simulink model "a"  (R2025b)
settings: Solver=VariableStepAuto  StartTime=0.0  StopTime=50  RelTol=1e-3
values from neighbouring files (symbols this model uses):
  Cd_mach = data_flight.CD    [load_aero.m]
  CnA_mach = data_flight.("CNalpha (0 to 4 deg) (per rad)")    [load_aero.m]
  Cp_inches_mach = data_flight.CP    [load_aero.m]
  Mach_vec = data_flight.Mach    [load_aero.m]
  thrust_force_vec = eng_data(:, 2)    [load_aero.m]
  thrust_time_vec = eng_data(:, 1)    [load_aero.m]
libraries: simulink_extras x6, aerolibasang x3, slpidlib x3, aerolibwind2 x2, aerolibanim x1, aerolibatmos2 x1, simulink x1
settings Model: Creator=anth  LastModifiedBy=anth

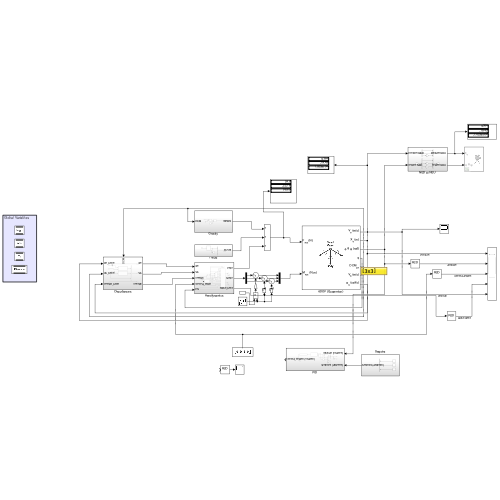
[thumbnail: Simulink's stored preview of the top-level diagram]
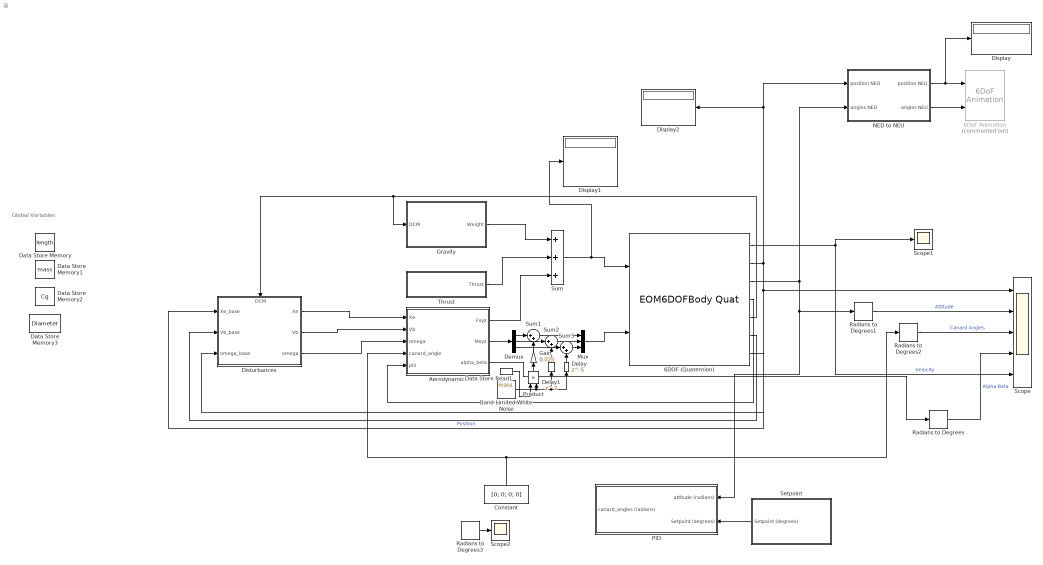
== system a ==
  note: Global Variables
  6DOF (Quaternion) : EOM6DOFBodyQuat  pm_0=[0.5 0.5 -0.5]  mass_0=5  inertia=[0.06 0 0; 0 0.06 0; 0 0 0.00056]
  6DoF Animation : aerolibanim/6DoF Animation  Commented=on  u1=[-4000 4000 -2000 2000 -5000000 4000000]  u2=0.1  u3=2  u4=[-1000 0 -1000]  u5=Fly alongside  u6=[40 5 -40]  u7=10  u8=on
  Aerodynamics : Subsystem
  Band-Limited White Noise : simulink/Sources/Band-Limited White Noise  Cov=[0.1]  Ts=0.1  seed=[23341]
  Constant : Constant  Value=[0; 0; 0; 0]
  Data Store Memory : DataStoreMemory  DataStoreName=length  WriteAfterWriteMsg=warning  InitialValue=1.524  ShowAdditionalParam=off
  Data Store Memory1 : DataStoreMemory  DataStoreName=mass  WriteAfterWriteMsg=warning  InitialValue=5  ShowAdditionalParam=off
  Data Store Memory2 : DataStoreMemory  DataStoreName=Cg  WriteAfterWriteMsg=warning  InitialValue=0.911682  ShowAdditionalParam=off
  Data Store Memory3 : DataStoreMemory  DataStoreName=Diameter  WriteAfterWriteMsg=warning  InitialValue=0.1016  ShowAdditionalParam=off
  Data Store Read1 : DataStoreRead  DataStoreName=mass  IndexOptions=Index vector (dialog)  Indices=1  OutputSizes=1
  Delay : Delay  DelayLength=5
  Delay1 : Delay
  Demux : Demux  Outputs=3
  Display : Display
  Display1 : Display
  Display2 : Display
  Disturbances : Subsystem
      settings: PortSchema="{\"entries\":[{\"content\":{\"sides\":[{\"content\":{\"connectorIds\":[\"In1\",\"In2\",\"In3\"]},\"type\":\"ConnectorPlacement.EquallySpacedRectSide\",\"uuid\":\"32f54cef-b4cb-4256-8316-c563039928ca\"},{\"content\":{\"connectorIds\":[\"Out1\",\"Out2\",\"Out3\"],\"side\":\"RIGHT\"},\"type\":\"ConnectorPlacement.EquallySpacedRectSide\",\"uuid\":\"bb564e65-4080-434d-8692-2d229c22ab5f\"},{\"content\":{\"connectorIds\":[\"In4\"],\"side\":\"TOP\"},\"type\":\"ConnectorPlacement.EquallySpacedRectSide\",\"uuid\":\"6318908c-0300-48fa-8f39-f8088bf31443\"}]},\"type\":\"ConnectorPlacement.EquallySpacedConnector\",\"uuid\":\"3467b8b9-b405-4e5c-95ab-dad331d67992\"}],\"packageUris\":[\"http://schema.mathworks.com/mf0/Connector/R2020b\"],\"version\":\"1.0\"}"
  Gain : Gain  Gain=0.025
  Gravity : Subsystem
  Mux : Mux  Inputs=3
  NED to NEU : Subsystem
  PID : Subsystem
  Product : Product
  Radians to Degrees{,1..3} (4 alike) : simulink_extras/Transformations/Radians to Degrees
  Scope : Scope  NumInputPorts=5
      settings: ActiveDisplayYMinimum=-186.34807824721173  ActiveDisplayYMaximum=22699.188645995033  DataLoggingVariableName=ScopeData7
  Scope1 : Scope
      settings: DataLoggingVariableName=ScopeData8
  Scope2 : Scope
      settings: ActiveDisplayYMinimum=-0.21482274425849368  ActiveDisplayYMaximum=0.19778218203879105  DataLoggingVariableName=ScopeData10
  Setpoint : Subsystem
  Sum : Sum  Inputs=+++
  Sum1 : Sum  Inputs=|++
  Sum2 : Sum  Inputs=|++
  Sum3 : Sum  Inputs=|++
  Thrust : Subsystem
  wires:
  Sum/1 -> Display1/1, 6DOF (Quaternion)/1
  Aerodynamics/1(Fxyz) -> Sum/3
  Aerodynamics/2(Mxyz) -> Demux/1
  Mux/1 -> 6DOF (Quaternion)/2
  Sum3/1 -> Mux/3
  Sum2/1 -> Mux/2
  Sum1/1 -> Mux/1
  Demux/1 -> Sum1/1
  Demux/2 -> Sum2/1
  Demux/3 -> Sum3/1
  Band-Limited White Noise/1 -> Product/2, Delay1/1, Delay/1
  Gain/1 -> Sum1/2
  Thrust/1(Thrust) -> Sum/2
  Gravity/1(Weight) -> Sum/1
  NED to NEU/1(position NEU) -> Display/1, 6DoF Animation/1
  NED to NEU/2(angles NEU) -> 6DoF Animation/2
  Setpoint/1(Setpoint (degrees)) -> PID/2(Setpoint (degrees))
  Disturbances/2(Vb) -> Aerodynamics/2(Vb)
  Disturbances/1(Xe) -> Aerodynamics/1(Xe)
  Disturbances/3(omega) -> Aerodynamics/3(omega)
  6DOF (Quaternion)/7 -> Disturbances/3(omega_base)
  6DOF (Quaternion)/6 -> Disturbances/2(Vb_base)
  6DOF (Quaternion)/2 -> NED to NEU/1(position NED), Display2/1, Scope/1, Disturbances/1(Xe_base)  "Position"
  6DOF (Quaternion)/5 -> Disturbances/4(DCM), Gravity/1(DCM)
  6DOF (Quaternion)/4 -> Aerodynamics/5(phi)
  Aerodynamics/3(alpha_beta) -> Radians to Degrees/1
  Radians to Degrees/1 -> Scope/4  "Alpha Beta"
  6DOF (Quaternion)/1 -> Scope/5, Scope1/1  "Velocity"
  Radians to Degrees1/1 -> Scope/2  "Attitude"
  6DOF (Quaternion)/3 -> NED to NEU/2(angles NED), PID/1(attitude (radians)), Radians to Degrees1/1
  Radians to Degrees2/1 -> Scope/3  "Canard Angles"
  Delay1/1 -> Sum2/2
  Delay/1 -> Sum3/2
  Radians to Degrees3/1 -> Scope2/1
  Constant/1 -> Radians to Degrees2/1, Aerodynamics/4(canard_angle)
  Product/1 -> Gain/1
  Data Store Read1/1 -> Product/1

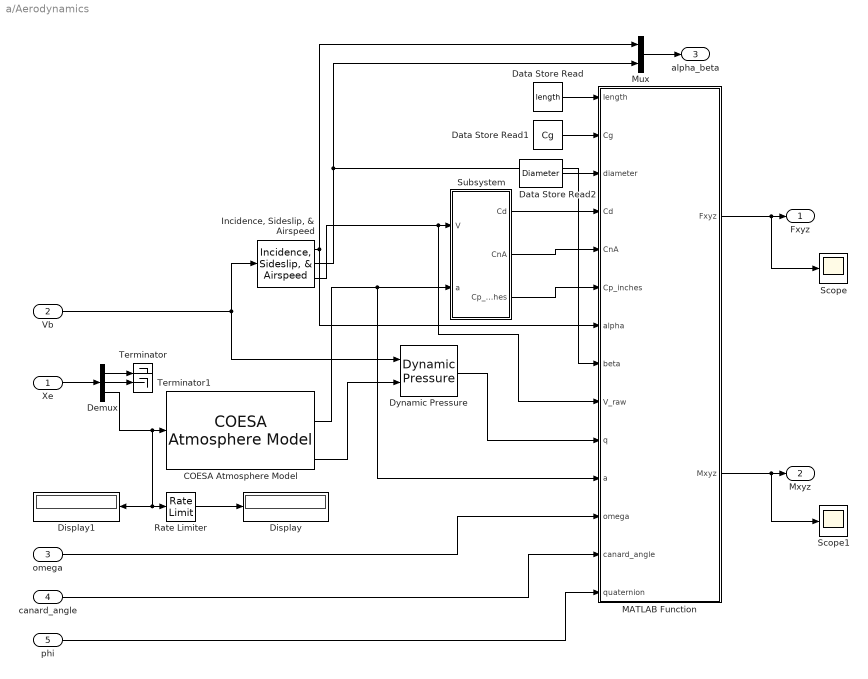
== system a/Aerodynamics ==
  Xe : Inport
  Vb : Inport  Port=2
  omega : Inport  Port=3
  canard_angle : Inport  Port=4
  phi : Inport  Port=5
  COESA Atmosphere Model : aerolibatmos2/COESA Atmosphere Model  units=Metric (MKS)  spec=1976 COESA-extended U.S. Standard Atmosphere  model=Profile  profile_var=High temperature  profile_percent=1%  profile_alt=5 km (16404 ft)  envelope_var=High temperature  envelope_percent=1%  action=Warning
  Data Store Read : DataStoreRead  DataStoreName=length  IndexOptions=Index vector (dialog)  Indices=1  OutputSizes=1
  Data Store Read1 : DataStoreRead  DataStoreName=Cg  IndexOptions=Index vector (dialog)  Indices=1  OutputSizes=1
  Data Store Read2 : DataStoreRead  DataStoreName=Diameter  IndexOptions=Index vector (dialog)  Indices=1  OutputSizes=1
  Demux : Demux  Outputs=3
  Display : Display
  Display1 : Display
  Dynamic Pressure : aerolibasang/Dynamic Pressure
  "Incidence, Sideslip, & Airspeed" : aerolibasang/Incidence, Sideslip, & Airspeed
  MATLAB Function : MATLAB Function  TreatAsAtomicUnit=on
  Mux : Mux  Inputs=2
  Rate Limiter : RateLimiter  RisingSlewLimit=inf  FallingSlewLimit=0  SampleTimeMode=inherited
  Scope : Scope
      settings: ActiveDisplayYMinimum=-4834.811497564544  ActiveDisplayYMaximum=1699.3324805277052
  Scope1 : Scope
      settings: DataLoggingVariableName=ScopeData2
  Subsystem : Subsystem
  Terminator : Terminator
  Terminator1 : Terminator
  Fxyz : Outport
  Mxyz : Outport  Port=2
  alpha_beta : Outport  Port=3
  wires:
  Xe/1 -> Demux/1
  Demux/1 -> Terminator/1
  Demux/2 -> Terminator1/1
  Demux/3 -> Display1/1, Rate Limiter/1, COESA Atmosphere Model/1
  Rate Limiter/1 -> Display/1
  COESA Atmosphere Model/4 -> Dynamic Pressure/2
  Vb/1 -> "Incidence, Sideslip, & Airspeed"/1, Dynamic Pressure/1
  "Incidence, Sideslip, & Airspeed"/3 -> MATLAB Function/9(V_raw), Subsystem/1(V)
  COESA Atmosphere Model/2 -> Subsystem/2(a), MATLAB Function/11(a)
  Mux/1 -> alpha_beta/1
  "Incidence, Sideslip, & Airspeed"/1 -> MATLAB Function/7(alpha), Mux/1
  "Incidence, Sideslip, & Airspeed"/2 -> MATLAB Function/8(beta), Mux/2
  MATLAB Function/1(Fxyz) -> Scope/1, Fxyz/1
  MATLAB Function/2(Mxyz) -> Scope1/1, Mxyz/1
  Subsystem/1(Cd) -> MATLAB Function/4(Cd)
  Subsystem/2(CnA) -> MATLAB Function/5(CnA)
  Subsystem/3(Cp_inches) -> MATLAB Function/6(Cp_inches)
  Dynamic Pressure/1 -> MATLAB Function/10(q)
  omega/1 -> MATLAB Function/12(omega)
  canard_angle/1 -> MATLAB Function/13(canard_angle)
  phi/1 -> MATLAB Function/14(quaternion)
  Data Store Read1/1 -> MATLAB Function/2(Cg)
  Data Store Read2/1 -> MATLAB Function/3(diameter)
  Data Store Read/1 -> MATLAB Function/1(length)

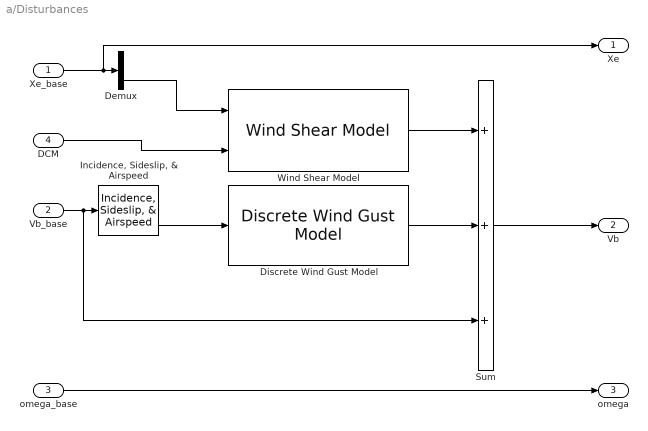
== system a/Disturbances ==
  Xe_base : Inport
  Vb_base : Inport  Port=2
  omega_base : Inport  Port=3
  DCM : Inport  Port=4
  Demux : Demux  Outputs=3
  Discrete Wind Gust Model : aerolibwind2/Discrete Wind Gust Model  units=Metric (MKS)  Gx=on  Gy=on  Gz=on  t_0=5  d_m=[120 120 80]  v_m=[3.5 3.5 3.0]
  "Incidence, Sideslip, & Airspeed" : aerolibasang/Incidence, Sideslip, & Airspeed
  Sum : Sum  Inputs=+++
  Wind Shear Model : aerolibwind2/Wind Shear Model  units=Metric (MKS)  phase=Category C - Terminal Flight Phase  W_20=15  Wdeg=0
  Xe : Outport
  Vb : Outport  Port=2
  omega : Outport  Port=3
  wires:
  omega_base/1 -> omega/1
  Vb_base/1 -> Sum/3, "Incidence, Sideslip, & Airspeed"/1
  "Incidence, Sideslip, & Airspeed"/3 -> Discrete Wind Gust Model/1
  Discrete Wind Gust Model/1 -> Sum/2
  Wind Shear Model/1 -> Sum/1
  Sum/1 -> Vb/1
  DCM/1 -> Wind Shear Model/2
  Demux/3 -> Wind Shear Model/1
  Xe_base/1 -> Xe/1, Demux/1

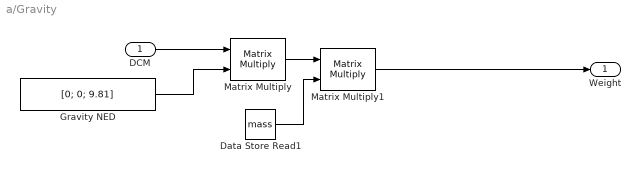
== system a/Gravity ==
  DCM : Inport
  Data Store Read1 : DataStoreRead  DataStoreName=mass  IndexOptions=Index vector (dialog)  Indices=1  OutputSizes=1
  Gravity NED : Constant  Value=[0; 0; 9.81]
  Matrix Multiply : Product  Multiplication=Matrix(*)
  Matrix Multiply1 : Product  Multiplication=Matrix(*)
  Weight : Outport
  wires:
  DCM/1 -> Matrix Multiply/1
  Gravity NED/1 -> Matrix Multiply/2
  Matrix Multiply1/1 -> Weight/1
  Data Store Read1/1 -> Matrix Multiply1/2
  Matrix Multiply/1 -> Matrix Multiply1/1

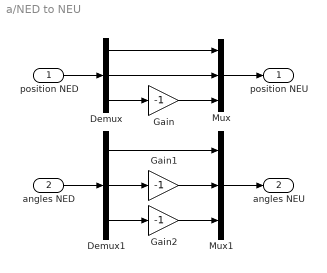
== system a/NED to NEU ==
  position NED : Inport
  angles NED : Inport  Port=2
  Demux : Demux  Outputs=3
  Demux1 : Demux  Outputs=3
  Gain : Gain  Gain=-1
  Gain1 : Gain  Gain=-1
  Gain2 : Gain  Gain=-1
  Mux : Mux  Inputs=3
  Mux1 : Mux  Inputs=3
  position NEU : Outport
  angles NEU : Outport  Port=2
  wires:
  Demux1/2 -> Gain1/1
  Demux1/3 -> Gain2/1
  Gain2/1 -> Mux1/3
  Gain1/1 -> Mux1/2
  Demux1/1 -> Mux1/1
  Demux/3 -> Gain/1
  Gain/1 -> Mux/3
  Demux/1 -> Mux/1
  Demux/2 -> Mux/2
  Mux1/1 -> angles NEU/1
  Mux/1 -> position NEU/1
  position NED/1 -> Demux/1
  angles NED/1 -> Demux1/1

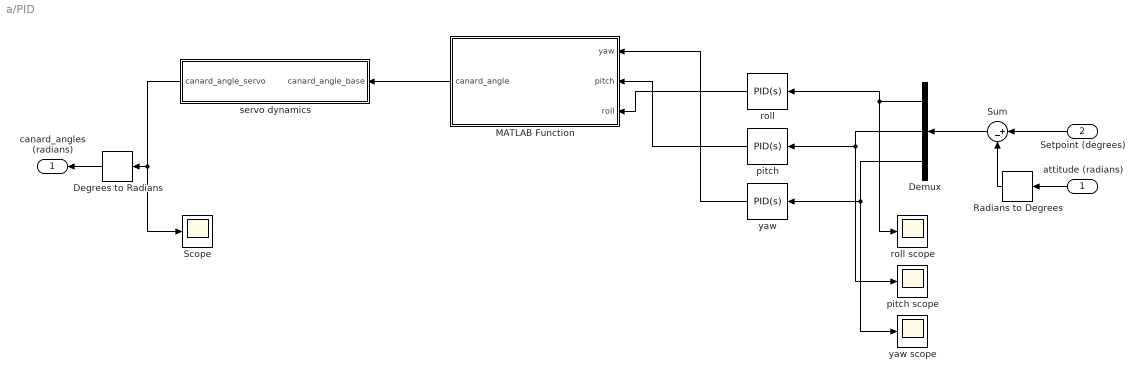
== system a/PID ==
  attitude (radians) : Inport
  Setpoint (degrees) : Inport  Port=2
  Degrees to Radians : simulink_extras/Transformations/Degrees to Radians
  Demux : Demux  Outputs=3
  MATLAB Function : MATLAB Function  TreatAsAtomicUnit=on
  Radians to Degrees : simulink_extras/Transformations/Radians to Degrees
  Scope : Scope
      settings: DataLoggingVariableName=ScopeData3
  Sum : Sum  Inputs=|+-
  pitch : slpidlib/PID Controller  Controller=PID  Form=Parallel  TimeDomain=Continuous-time  UseExternalTs=off  SampleTime=-1  IntegratorMethod=Forward Euler  FilterMethod=Forward Euler  ControllerParametersSource=internal  P=1.1  I=0.8  UseKiTs=off  D=0.05  UseExternalDerivativeSource=off  N=100  UseFilter=on  TunerSelectOption=Transfer Function Based (PID Tuner App)  InitialConditionSource=internal  InitialConditionForIntegrator=0  InitialConditionForFilter=0  DifferentiatorICPrevScaledInput=0  ExternalReset=none  TrackingMode=off  Kt=1  LimitOutput=off  SatLimitsSource=internal  UpperSaturationLimit=inf  LowerSaturationLimit=-inf  LinearizeAsGain=on  AntiWindupMode=none  Kb=1  LimitIntegrator=off  UpperIntegratorSaturationLimit=inf  LowerIntegratorSaturationLimit=-inf  POutMin=[]  POutMax=[]  IOutMin=[]  IOutMax=[]  DOutMin=[]  DOutMax=[]  NOutMin=[]  NOutMax=[]  SumOutMin=[]  SumOutMax=[]  SaturationOutMin=[]  SaturationOutMax=[]  PParamMin=[]  PParamMax=[]  IParamMin=[]  IParamMax=[]  DParamMin=[]  DParamMax=[]  NParamMin=[]  NParamMax=[]  KbParamMin=[]  KbParamMax=[]  KtParamMin=[]  KtParamMax=[]  KbOutMin=[]  KbOutMax=[]  KtOutMin=[]  KtOutMax=[]  IntegratorOutMin=[]  IntegratorOutMax=[]  FilterOutMin=[]  FilterOutMax=[]  SumI1OutMin=[]  SumI1OutMax=[]  SumI2OutMin=[]  SumI2OutMax=[]  SumI3OutMin=[]  SumI3OutMax=[]  SumI4OutMin=[]  SumI4OutMax=[]  SumDOutMin=[]  SumDOutMax=[]  DifferentiatorOutMin=[]  DifferentiatorOutMax=[]  FilterDiffOutCoefMin=[]  FilterDiffOutCoefMax=[]  ReciprocalOutMin=[]  ReciprocalOutMax=[]  SumDenOutMin=[]  SumDenOutMax=[]  SumNumOutMin=[]  SumNumOutMax=[]  DivideOutMin=[]  DivideOutMax=[]  UdiffTsProdOutMin=[]  UdiffTsProdOutMax=[]  NTsProdOutMin=[]  NTsProdOutMax=[]  UintegralTsProdOutMin=[]  UintegralTsProdOutMax=[]  UngainTsProdOutMin=[]  UngainTsProdOutMax=[]  ClampingZeroOutDataTypeStr=Inherit: Inherit via back propagation  ClampingZeroOutMin=[]  ClampingZeroOutMax=[]  FilterDenConstantOutDataTypeStr=Inherit: Inherit via back propagation  FilterDenConstantOutMin=[]  FilterDenConstantOutMax=[]  PCopyOutDataTypeStr=Inherit: Inherit via back propagation  PCopyOutMin=[]  PCopyOutMax=[]  NCopyOutDataTypeStr=Inherit: Inherit via back propagation  NCopyOutMin=[]  NCopyOutMax=[]  IntegratorContinuousStateAttributes=''  IntegratorStateMustResolveToSignalObject=off  IntegratorRTWStateStorageClass=Auto  FilterContinuousStateAttributes=''  FilterStateMustResolveToSignalObject=off  FilterRTWStateStorageClass=Auto  ParallelPVariant=InternalParameters  IdealPVariant=Disabled  IVariant=InternalParameters  DVariant=InternalParameters  IntegratorVariant=Continuous  SatVariant=Disabled  AWVariant=Passthrough  PCopyVariant=Disabled  TRVariant=Disabled  FdbkBlocksVariant=Forward  IdealPFdbkVariant=Disabled  SatFdbkVariant=Disabled  DerivativeFilterVariant=ContFilter  NVariant=InternalParameters  NCopyVariant=Disabled  FilterICVariant=InternalICsFilter  IntegratorICVariant=InternalICs  ExternalResetVariant=Disabled  TRSumVariant=Passthrough  SumFdbkVariant=Disabled  SumVariant=Sum_PID  TsampFilterVariant=InternalTs  TsampNgainVariant=Passthrough  TsampIntegralVariant=Disabled_SignalSpec  ExternalSaturationOutDataTypeStr=Inherit: Same as second input  DerivativeSourceVariant=ErrorSignal  PreIntVariant=InternalPreInt
  pitch scope : Scope
      settings: DataLoggingVariableName=ScopeData5
  roll : slpidlib/PID Controller  Controller=PID  Form=Parallel  TimeDomain=Continuous-time  UseExternalTs=off  SampleTime=-1  IntegratorMethod=Forward Euler  FilterMethod=Forward Euler  ControllerParametersSource=internal  P=0.06  I=0.0005  UseKiTs=off  D=0.02  UseExternalDerivativeSource=off  N=100  UseFilter=on  TunerSelectOption=Transfer Function Based (PID Tuner App)  InitialConditionSource=internal  InitialConditionForIntegrator=0  InitialConditionForFilter=0  DifferentiatorICPrevScaledInput=0  ExternalReset=none  TrackingMode=off  Kt=1  LimitOutput=off  SatLimitsSource=internal  UpperSaturationLimit=inf  LowerSaturationLimit=-inf  LinearizeAsGain=on  AntiWindupMode=none  Kb=1  LimitIntegrator=off  UpperIntegratorSaturationLimit=inf  LowerIntegratorSaturationLimit=-inf  POutMin=[]  POutMax=[]  IOutMin=[]  IOutMax=[]  DOutMin=[]  DOutMax=[]  NOutMin=[]  NOutMax=[]  SumOutMin=[]  SumOutMax=[]  SaturationOutMin=[]  SaturationOutMax=[]  PParamMin=[]  PParamMax=[]  IParamMin=[]  IParamMax=[]  DParamMin=[]  DParamMax=[]  NParamMin=[]  NParamMax=[]  KbParamMin=[]  KbParamMax=[]  KtParamMin=[]  KtParamMax=[]  KbOutMin=[]  KbOutMax=[]  KtOutMin=[]  KtOutMax=[]  IntegratorOutMin=[]  IntegratorOutMax=[]  FilterOutMin=[]  FilterOutMax=[]  SumI1OutMin=[]  SumI1OutMax=[]  SumI2OutMin=[]  SumI2OutMax=[]  SumI3OutMin=[]  SumI3OutMax=[]  SumI4OutMin=[]  SumI4OutMax=[]  SumDOutMin=[]  SumDOutMax=[]  DifferentiatorOutMin=[]  DifferentiatorOutMax=[]  FilterDiffOutCoefMin=[]  FilterDiffOutCoefMax=[]  ReciprocalOutMin=[]  ReciprocalOutMax=[]  SumDenOutMin=[]  SumDenOutMax=[]  SumNumOutMin=[]  SumNumOutMax=[]  DivideOutMin=[]  DivideOutMax=[]  UdiffTsProdOutMin=[]  UdiffTsProdOutMax=[]  NTsProdOutMin=[]  NTsProdOutMax=[]  UintegralTsProdOutMin=[]  UintegralTsProdOutMax=[]  UngainTsProdOutMin=[]  UngainTsProdOutMax=[]  ClampingZeroOutDataTypeStr=Inherit: Inherit via back propagation  ClampingZeroOutMin=[]  ClampingZeroOutMax=[]  FilterDenConstantOutDataTypeStr=Inherit: Inherit via back propagation  FilterDenConstantOutMin=[]  FilterDenConstantOutMax=[]  PCopyOutDataTypeStr=Inherit: Inherit via back propagation  PCopyOutMin=[]  PCopyOutMax=[]  NCopyOutDataTypeStr=Inherit: Inherit via back propagation  NCopyOutMin=[]  NCopyOutMax=[]  IntegratorContinuousStateAttributes=''  IntegratorStateMustResolveToSignalObject=off  IntegratorRTWStateStorageClass=Auto  FilterContinuousStateAttributes=''  FilterStateMustResolveToSignalObject=off  FilterRTWStateStorageClass=Auto  ParallelPVariant=InternalParameters  IdealPVariant=Disabled  IVariant=InternalParameters  DVariant=InternalParameters  IntegratorVariant=Continuous  SatVariant=Disabled  AWVariant=Passthrough  PCopyVariant=Disabled  TRVariant=Disabled  FdbkBlocksVariant=Forward  IdealPFdbkVariant=Disabled  SatFdbkVariant=Disabled  DerivativeFilterVariant=ContFilter  NVariant=InternalParameters  NCopyVariant=Disabled  FilterICVariant=InternalICsFilter  IntegratorICVariant=InternalICs  ExternalResetVariant=Disabled  TRSumVariant=Passthrough  SumFdbkVariant=Disabled  SumVariant=Sum_PID  TsampFilterVariant=InternalTs  TsampNgainVariant=Passthrough  TsampIntegralVariant=Disabled_SignalSpec  ExternalSaturationOutDataTypeStr=Inherit: Same as second input  DerivativeSourceVariant=ErrorSignal  PreIntVariant=InternalPreInt
  roll scope : Scope
      settings: DataLoggingVariableName=ScopeData4
  servo dynamics : Subsystem
  yaw : slpidlib/PID Controller  Controller=PID  Form=Parallel  TimeDomain=Continuous-time  UseExternalTs=off  SampleTime=-1  IntegratorMethod=Forward Euler  FilterMethod=Forward Euler  ControllerParametersSource=internal  P=1.1  I=0.8  UseKiTs=off  D=0.05  UseExternalDerivativeSource=off  N=100  UseFilter=on  TunerSelectOption=Transfer Function Based (PID Tuner App)  InitialConditionSource=internal  InitialConditionForIntegrator=0  InitialConditionForFilter=0  DifferentiatorICPrevScaledInput=0  ExternalReset=none  TrackingMode=off  Kt=1  LimitOutput=on  SatLimitsSource=internal  UpperSaturationLimit=10  LowerSaturationLimit=-10  LinearizeAsGain=on  AntiWindupMode=back-calculation  Kb=1  LimitIntegrator=off  UpperIntegratorSaturationLimit=inf  LowerIntegratorSaturationLimit=-inf  POutMin=[]  POutMax=[]  IOutMin=[]  IOutMax=[]  DOutMin=[]  DOutMax=[]  NOutMin=[]  NOutMax=[]  SumOutMin=[]  SumOutMax=[]  SaturationOutMin=[]  SaturationOutMax=[]  PParamMin=[]  PParamMax=[]  IParamMin=[]  IParamMax=[]  DParamMin=[]  DParamMax=[]  NParamMin=[]  NParamMax=[]  KbParamMin=[]  KbParamMax=[]  KtParamMin=[]  KtParamMax=[]  KbOutMin=[]  KbOutMax=[]  KtOutMin=[]  KtOutMax=[]  IntegratorOutMin=[]  IntegratorOutMax=[]  FilterOutMin=[]  FilterOutMax=[]  SumI1OutMin=[]  SumI1OutMax=[]  SumI2OutMin=[]  SumI2OutMax=[]  SumI3OutMin=[]  SumI3OutMax=[]  SumI4OutMin=[]  SumI4OutMax=[]  SumDOutMin=[]  SumDOutMax=[]  DifferentiatorOutMin=[]  DifferentiatorOutMax=[]  FilterDiffOutCoefMin=[]  FilterDiffOutCoefMax=[]  ReciprocalOutMin=[]  ReciprocalOutMax=[]  SumDenOutMin=[]  SumDenOutMax=[]  SumNumOutMin=[]  SumNumOutMax=[]  DivideOutMin=[]  DivideOutMax=[]  UdiffTsProdOutMin=[]  UdiffTsProdOutMax=[]  NTsProdOutMin=[]  NTsProdOutMax=[]  UintegralTsProdOutMin=[]  UintegralTsProdOutMax=[]  UngainTsProdOutMin=[]  UngainTsProdOutMax=[]  ClampingZeroOutDataTypeStr=Inherit: Inherit via back propagation  ClampingZeroOutMin=[]  ClampingZeroOutMax=[]  FilterDenConstantOutDataTypeStr=Inherit: Inherit via back propagation  FilterDenConstantOutMin=[]  FilterDenConstantOutMax=[]  PCopyOutDataTypeStr=Inherit: Inherit via back propagation  PCopyOutMin=[]  PCopyOutMax=[]  NCopyOutDataTypeStr=Inherit: Inherit via back propagation  NCopyOutMin=[]  NCopyOutMax=[]  IntegratorContinuousStateAttributes=''  IntegratorStateMustResolveToSignalObject=off  IntegratorRTWStateStorageClass=Auto  FilterContinuousStateAttributes=''  FilterStateMustResolveToSignalObject=off  FilterRTWStateStorageClass=Auto  ParallelPVariant=InternalParameters  IdealPVariant=Disabled  IVariant=InternalParameters  DVariant=InternalParameters  IntegratorVariant=Continuous  SatVariant=Enabled  AWVariant=BackCalculation  PCopyVariant=Disabled  TRVariant=Disabled  FdbkBlocksVariant=Forward  IdealPFdbkVariant=Disabled  SatFdbkVariant=Disabled  DerivativeFilterVariant=ContFilter  NVariant=InternalParameters  NCopyVariant=Disabled  FilterICVariant=InternalICsFilter  IntegratorICVariant=InternalICs  ExternalResetVariant=Disabled  TRSumVariant=Passthrough  SumFdbkVariant=Disabled  SumVariant=Sum_PID  TsampFilterVariant=InternalTs  TsampNgainVariant=Passthrough  TsampIntegralVariant=Disabled_SignalSpec  ExternalSaturationOutDataTypeStr=Inherit: Same as second input  DerivativeSourceVariant=ErrorSignal  PreIntVariant=InternalPreInt
  yaw scope : Scope
      settings: DataLoggingVariableName=ScopeData6
  canard_angles (radians) : Outport
  wires:
  Degrees to Radians/1 -> canard_angles (radians)/1
  servo dynamics/1(canard_angle_servo) -> Scope/1, Degrees to Radians/1
  MATLAB Function/1(canard_angle) -> servo dynamics/1(canard_angle_base)
  Setpoint (degrees)/1 -> Sum/1
  attitude (radians)/1 -> Radians to Degrees/1
  Radians to Degrees/1 -> Sum/2
  Sum/1 -> Demux/1
  Demux/3 -> yaw scope/1, yaw/1
  Demux/2 -> pitch scope/1, pitch/1
  Demux/1 -> roll/1, roll scope/1
  yaw/1 -> MATLAB Function/1(yaw)
  pitch/1 -> MATLAB Function/2(pitch)
  roll/1 -> MATLAB Function/3(roll)

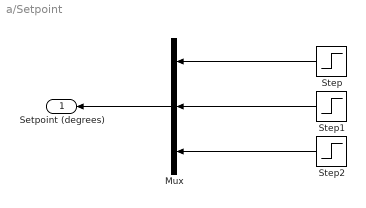
== system a/Setpoint ==
  Mux : Mux  Inputs=3
  Step : Step  SampleTime=0
  Step1 : Step  Before=1  After=0  SampleTime=0
  Step2 : Step  Before=1  After=0  SampleTime=0
  Setpoint (degrees) : Outport
  wires:
  Mux/1 -> Setpoint (degrees)/1
  Step/1 -> Mux/1
  Step1/1 -> Mux/2
  Step2/1 -> Mux/3

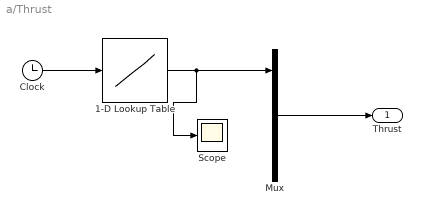
== system a/Thrust ==
  1-D Lookup Table : Lookup_n-D  NumberOfTableDimensions=1  BreakpointsForDimension1=thrust_time_vec  Table=thrust_force_vec  ExtrapMethod=Clip  InternalRulePriority=Speed  RndMeth=Simplest
  Clock : Clock
  Mux : Mux  Inputs=3
  Scope : Scope
      settings: ActiveDisplayYMinimum=-249.40858631973464  ActiveDisplayYMaximum=1239.3394316516465  DataLoggingVariableName=ScopeData9
  Thrust : Outport
  wires:
  1-D Lookup Table/1 -> Scope/1, Mux/1
  Mux/1 -> Thrust/1
  Clock/1 -> 1-D Lookup Table/1

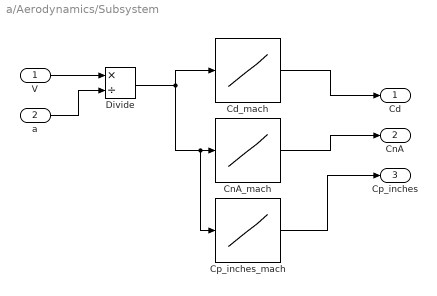
== system a/Aerodynamics/Subsystem ==
  V : Inport
  a : Inport  Port=2
  Cd_mach : Lookup_n-D  NumberOfTableDimensions=1  BreakpointsForDimension1=Mach_vec  Table=Cd_mach  InternalRulePriority=Speed  RndMeth=Simplest
  CnA_mach : Lookup_n-D  NumberOfTableDimensions=1  BreakpointsForDimension1=Mach_vec  Table=CnA_mach  InternalRulePriority=Speed  RndMeth=Simplest
  Cp_inches_mach : Lookup_n-D  NumberOfTableDimensions=1  BreakpointsForDimension1=Mach_vec  Table=Cp_inches_mach  InternalRulePriority=Speed  RndMeth=Simplest
  Divide : Product  Inputs=*/
  Cd : Outport
  CnA : Outport  Port=2
  Cp_inches : Outport  Port=3
  wires:
  V/1 -> Divide/1
  a/1 -> Divide/2
  Cp_inches_mach/1 -> Cp_inches/1
  CnA_mach/1 -> CnA/1
  Cd_mach/1 -> Cd/1
  Divide/1 -> Cp_inches_mach/1, CnA_mach/1, Cd_mach/1

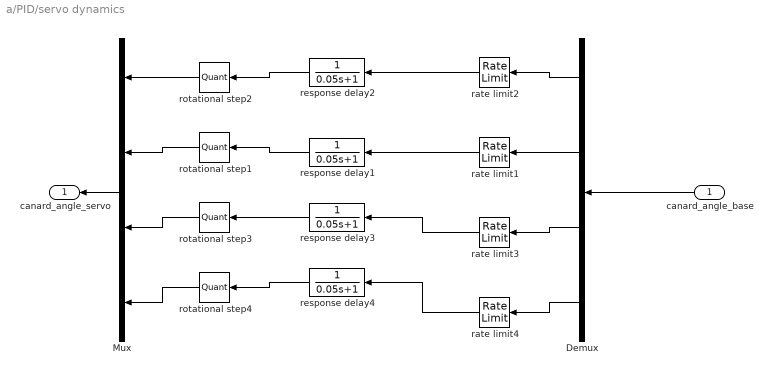
== system a/PID/servo dynamics ==
  canard_angle_base : Inport
  Demux : Demux
  Mux : Mux
  rate limit{1..4} (4 alike) : RateLimiter  RisingSlewLimit=80  FallingSlewLimit=-80  SampleTimeMode=inherited
  response delay{1..4} (4 alike) : TransferFcn  Denominator=[0.05 1]
  rotational step{1..4} (4 alike) : Quantizer  QuantizationInterval=0.2
  canard_angle_servo : Outport
  wires:
  Mux/1 -> canard_angle_servo/1
  canard_angle_base/1 -> Demux/1
  Demux/1 -> rate limit2/1
  Demux/2 -> rate limit1/1
  Demux/3 -> rate limit3/1
  Demux/4 -> rate limit4/1
  rotational step2/1 -> Mux/1
  rotational step1/1 -> Mux/2
  rotational step3/1 -> Mux/3
  rotational step4/1 -> Mux/4
  rate limit2/1 -> response delay2/1
  rate limit1/1 -> response delay1/1
  rate limit3/1 -> response delay3/1
  rate limit4/1 -> response delay4/1
  response delay4/1 -> rotational step4/1
  response delay3/1 -> rotational step3/1
  response delay1/1 -> rotational step1/1
  response delay2/1 -> rotational step2/1

== matlab function a/PID/MATLAB Function ==
  data: yaw input; canard_angle output; pitch input; roll input
function canard_angle = mixer(yaw, pitch, roll)
% Cruciform canard mixer with roll-frame compensation
% Fin numbering clockwise: top=1, right=2, bottom=3, left=4
% Deflections defined in body axis frame (aero convention)
%
% Pitch/yaw demands rotated from world into body frame before mixing:
%   [p_b]   [ cos(roll)  sin(roll)] [pitch]
%   [y_b] = [-sin(roll)  cos(roll)] [yaw  ]
%
% Ref: Blakelock, Automatic Control of Aircraft and Missiles, Wiley 1991

limit = 10; %Prevents entering stall behaviour that is not modelled.

% Rotate world-frame demands into body frame
p_b =  pitch * cos(roll) + yaw * sin(roll);
y_b = -pitch * sin(roll) + yaw * cos(roll);

% Original mixing with body-frame demands substituted in
F1 =  roll - y_b;
F2 =  roll + p_b;
F3 = -roll - y_b;
F4 = -roll + p_b;

canard_angle = max(-limit, min(limit, [F1; F2; F3; F4]));
end

== matlab function a/Aerodynamics/MATLAB Function ==
  data: length input; Fxyz output; Cg input; diameter input; Cd input; CnA input; Cp_inches input; alpha input; beta input; V_raw input; q input; a input; omega input; canard_angle input; quaternion input; Mxyz output
function [Fxyz, Mxyz] = aerodynamics(length, Cg, diameter, Cd, CnA, Cp_inches, alpha,beta, V_raw, q, a, omega, canard_angle, quaternion)

%User Variables
Cmq = -10.0;    % Pitch damping derivative
Cnr = -10.0;    % Yaw damping derivative
Clp = -1.0;     % Roll damping derivative

p_rate = omega(1);      % Roll rate (rad/s)
q_rate = omega(2);      % Pitch rate (rad/s)
r_rate = omega(3);      % Yaw rate (rad/s)

phi_roll = atan2(2*(quaternion(1)*quaternion(2) + quaternion(3)*quaternion(4)), 1 - 2*(quaternion(2)^2 + quaternion(3)^2));

%System Varaibles
A_Ref = ((diameter/2)^2 * pi);
V = max(V_raw, 0.1);
Cp = (Cp_inches * 0.0254);
moment_arm = Cp - Cg;

Cn_alpha = CnA * sin(alpha);
Cn_beta = CnA * sin(beta);

p_hat = p_rate * diameter / (2*V);
q_hat = q_rate * length / (2*V);
r_hat = r_rate * length / (2*V);

%Forces
Fx_base = -q * A_Ref * Cd;
Fy_base = -q * A_Ref * Cn_beta;
Fz_base = -q * A_Ref * Cn_alpha;

Fxyz_base = [Fx_base; Fy_base; Fz_base];

%Moments
Mx_P_base = 0;
My_P_base = Fz_base * moment_arm;
Mz_P_base = -Fy_base * moment_arm;

Mx_D_base = q * A_Ref * Clp * diameter * p_hat;
My_D_base = q * A_Ref * Cmq * length * q_hat;
Mz_D_base = q * A_Ref * Cnr * length * r_hat;

Mx_base = Mx_P_base + Mx_D_base;
My_base = My_P_base + My_D_base;
Mz_base = Mz_P_base + Mz_D_base;

Mxyz_base = [Mx_base; My_base; Mz_base];

%===================================================

%Canards

%User Variables
Cp_canards = 0.266; %distance from tip to canards
canard_span = 0.16; %tip-to-tip distance
canard_area = 0.001; %m^2
moment_arm_canards = Cp_canards - Cg;
e = 0.8; %oswald efficiency factor (0.7 - 0.9) for canard Cd
canard_base_Cd = 0.02; %estimate for base drap

%System Variables
mach = V/a;
AR = (canard_span^2) / canard_area;
canard_radial_moment_arm = (canard_span - diameter)*0.25 + (diameter/2);

if mach < 0.9
    Beta_comp = sqrt(max(1-(mach^2), 0.01));
else
    Beta_comp = sqrt(max((mach^2) -1, 0.01));
end

% Roll-corrected local AoA per fin pair (Nielsen 1960)
% phi measured from RIGHT fin (fin 2), clockwise from front
phi_2 = 0;   phi_4 = pi;     % RIGHT/LEFT pair
phi_1 = 3*pi/2; phi_3 = pi/2; % TOP/DOWN pair

alpha_local_2 = alpha*cos(phi_2 - phi_roll) + beta*sin(phi_2 - phi_roll);
alpha_local_4 = alpha*cos(phi_4 - phi_roll) + beta*sin(phi_4 - phi_roll);
alpha_local_1 = alpha*cos(phi_1 - phi_roll) + beta*sin(phi_1 - phi_roll);
alpha_local_3 = alpha*cos(phi_3 - phi_roll) + beta*sin(phi_3 - phi_roll);

% Effective angles including canard deflection
eff_24 = ((canard_angle(2)+canard_angle(4))/2) - (alpha_local_2 - alpha_local_4)/2;
eff_13 = ((canard_angle(1)+canard_angle(3))/2) + (alpha_local_3 - alpha_local_1)/2;

CnA_canards = (2 * pi * AR) / (2 + sqrt(4 + (AR*Beta_comp)^2));

Cd_canard_1 = (CnA_canards * sin(canard_angle(1) + alpha_local_1))^2 / (pi * AR * e);
Cd_canard_2 = (CnA_canards * sin(canard_angle(2) + alpha_local_2))^2 / (pi * AR * e);
Cd_canard_3 = (CnA_canards * sin(canard_angle(3) + alpha_local_3))^2 / (pi * AR * e);
Cd_canard_4 = (CnA_canards * sin(canard_angle(4) + alpha_local_4))^2 / (pi * AR * e);

Cd_canards = ((Cd_canard_1 + Cd_canard_2 + Cd_canard_3 + Cd_canard_4)/4) + canard_base_Cd; %sum of all fin Cd/4 + base
if mach < 0.8 %Supersonic correction
    Cd_canards = Cd_canards / sqrt(1 - mach^2);
elseif mach >= 0.8 && mach < 1.2
    Cd_canards = Cd_canards * 2.5;
else
    Cd_canards = Cd_canards * 2.0;
end

roll_deflection = (canard_angle(1) + canard_angle(2) - canard_angle(3) - canard_angle(4))/4;

%Forces
Fx_canards = -q * canard_area * Cd_canards * 4;
Fy_canards = -q * canard_area * CnA_canards * sin(eff_13) * 2;
Fz_canards = -q * canard_area * CnA_canards * sin(eff_24) * 2;

Fxyz_canards = [Fx_canards; Fy_canards; Fz_canards];

%Moments
Mx_canards = q * canard_area * CnA_canards * roll_deflection * canard_radial_moment_arm * 4;
My_canards = Fz_canards * moment_arm_canards;
Mz_canards = -Fy_canards * moment_arm_canards;

%Damping is unnecessary for canards as it can just be included in base coefficients.

Mxyz_canards = [Mx_canards; My_canards; Mz_canards];




%===================================================



%Final Forces
Fxyz = Fxyz_base + Fxyz_canards;

%Final Moments
if V < 0.1
    Mxyz = [0; 0; 0];
else
    Mxyz = Mxyz_base + Mxyz_canards;
end
